simulink model "HapticPaddle_vR2018b"  (R2025a)
settings: Solver=FixedStepAuto  StartTime=0.0  StopTime=10  FixedStep=0.0001  RelTol=1e-3  EnableMultiTasking=on
values from neighbouring files (symbols this model uses):
  B_eq = B_p + R^2*B_m    (= 0.00017775)    [main.m]
  g = 9.81    [main.m]
  J_eq = (J_p + R^2*(J_rotor + J_m))    (= 0.000485304)    [main.m]
  l = 0.0251    [main.m]
  m_p = 0.048    [main.m]
  phi_target = 10.00    (= 10)    [main.m]
  R = r_p1 / r_m    (= 15)    [main.m]
  r_p2 = 0.081    [main.m]
  Tau_f_dry = 0.00156    [main.m]
libraries: simulink_extras x3, slpidlib x1
settings Model: Creator=jemetzge  LastModifiedBy=tk
settings SolverCC: AlgebraicLoopSolver=TrustRegion
settings DataIOCC: LimitDataPoints=on  SaveFormat=Array  SignalLoggingSaveFormat=ModelDataLogs  ReturnWorkspaceOutputs=off
settings OptimizationCC: ExpressionDepthLimit=2147483647.0  LifeSpan=inf
settings DebuggingCC: UnderspecifiedInitializationDetection=Classic  MergeDetectMultiDrivingBlocksExec=none  SolverPrmCheckMsg=warning  FcnCallInpInsideContextMsg=warning  UnconnectedInputMsg=warning  UnconnectedOutputMsg=warning  UnconnectedLineMsg=warning  StateNameClashWarn=warning  SFUnexpectedBacktrackingDiag=warning  SFNoUnconditionalDefaultTransitionDiag=warning  SFExecutionAtInitializationDiag=none  ArithmeticOperatorsInVariantConditions=warning
settings HardwareCC: ProdBitPerPointer=32.0  ProdBitPerSizeT=32.0  ProdBitPerPtrDiffT=32.0  ProdLargestAtomicFloat=None  ProdIntDivRoundTo=Undefined  ProdEndianess=Unspecified  ProdWordSize=32.0  ProdHWDeviceType=32-bit Generic
settings ModelReferenceCC: EnableRefExpFcnMdlSchedulingChecks=on  PropagateSignalLabelsOutOfModel=off
settings SFSimCC: SimUseLocalCustomCode=off  CustomCodeUndefinedFunction=UseInterfaceOnly
settings RTWCC: RTWUseLocalCustomCode=off  GPUComputeCapability=3.5  DLArmComputeVersion=19.05
settings CodeAppCC: StateflowObjectComments=on
settings GRTTargetCC: TargetLangStandard=C89/C90 (ANSI)  CombineOutputUpdateFcns=off  GRTInterface=on
settings ConfigComp: CovMetricSettings=dw  CovSaveCumulativeToWorkspaceVar=on  CovSaveSingleToWorkspaceVar=on  CovExternalEMLEnable=off  CovSFcnEnable=off

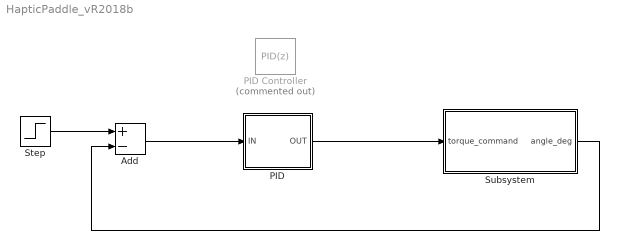
== system HapticPaddle_vR2018b ==
  Add : Sum  Inputs=+-
  PID : Subsystem
  PID Controller : slpidlib/PID Controller  Commented=on  Controller=PID  Form=Parallel  TimeDomain=Discrete-time  UseExternalTs=off  SampleTime=-1  IntegratorMethod=Forward Euler  FilterMethod=Forward Euler  ControllerParametersSource=internal  P=5  I=1  UseKiTs=off  D=5  UseExternalDerivativeSource=off  N=100  UseFilter=on  TunerSelectOption=Transfer Function Based (PID Tuner App)  InitialConditionSource=internal  InitialConditionForIntegrator=0  InitialConditionForFilter=0  DifferentiatorICPrevScaledInput=0  ExternalReset=none  TrackingMode=off  Kt=1  LimitOutput=off  SatLimitsSource=internal  UpperSaturationLimit=inf  LowerSaturationLimit=-inf  LinearizeAsGain=on  AntiWindupMode=none  Kb=1  LimitIntegrator=off  UpperIntegratorSaturationLimit=inf  LowerIntegratorSaturationLimit=-inf  POutMin=[]  POutMax=[]  IOutMin=[]  IOutMax=[]  DOutMin=[]  DOutMax=[]  NOutMin=[]  NOutMax=[]  SumOutMin=[]  SumOutMax=[]  SaturationOutMin=[]  SaturationOutMax=[]  PParamMin=[]  PParamMax=[]  IParamMin=[]  IParamMax=[]  DParamMin=[]  DParamMax=[]  NParamMin=[]  NParamMax=[]  KbParamMin=[]  KbParamMax=[]  KtParamMin=[]  KtParamMax=[]  KbOutMin=[]  KbOutMax=[]  KtOutMin=[]  KtOutMax=[]  IntegratorOutMin=[]  IntegratorOutMax=[]  FilterOutMin=[]  FilterOutMax=[]  SumI1OutMin=[]  SumI1OutMax=[]  SumI2OutMin=[]  SumI2OutMax=[]  SumI3OutMin=[]  SumI3OutMax=[]  SumI4OutMin=[]  SumI4OutMax=[]  SumDOutMin=[]  SumDOutMax=[]  DifferentiatorOutMin=[]  DifferentiatorOutMax=[]  FilterDiffOutCoefMin=[]  FilterDiffOutCoefMax=[]  ReciprocalOutMin=[]  ReciprocalOutMax=[]  SumDenOutMin=[]  SumDenOutMax=[]  SumNumOutMin=[]  SumNumOutMax=[]  DivideOutMin=[]  DivideOutMax=[]  UdiffTsProdOutMin=[]  UdiffTsProdOutMax=[]  NTsProdOutMin=[]  NTsProdOutMax=[]  UintegralTsProdOutMin=[]  UintegralTsProdOutMax=[]  UngainTsProdOutMin=[]  UngainTsProdOutMax=[]  ClampingZeroOutDataTypeStr=Inherit: Inherit via back propagation  ClampingZeroOutMin=[]  ClampingZeroOutMax=[]  FilterDenConstantOutDataTypeStr=Inherit: Inherit via back propagation  FilterDenConstantOutMin=[]  FilterDenConstantOutMax=[]  PCopyOutDataTypeStr=Inherit: Inherit via back propagation  PCopyOutMin=[]  PCopyOutMax=[]  NCopyOutDataTypeStr=Inherit: Inherit via back propagation  NCopyOutMin=[]  NCopyOutMax=[]  IntegratorContinuousStateAttributes=''  IntegratorStateMustResolveToSignalObject=off  IntegratorRTWStateStorageClass=Auto  FilterContinuousStateAttributes=''  FilterStateMustResolveToSignalObject=off  FilterRTWStateStorageClass=Auto  ParallelPVariant=InternalParameters  IdealPVariant=Disabled  IVariant=InternalParameters  DVariant=InternalParameters  IntegratorVariant=Discrete  SatVariant=Disabled  AWVariant=Passthrough  PCopyVariant=Disabled  TRVariant=Disabled  FdbkBlocksVariant=Forward  IdealPFdbkVariant=Disabled  SatFdbkVariant=Disabled  DerivativeFilterVariant=ForwardEulerFilter  NVariant=InternalParameters  NCopyVariant=Disabled  FilterICVariant=InternalICsFilter  IntegratorICVariant=InternalICs  ExternalResetVariant=Disabled  TRSumVariant=Passthrough  SumFdbkVariant=Disabled  SumVariant=Sum_PID  TsampFilterVariant=InternalTs  TsampNgainVariant=Passthrough  TsampIntegralVariant=Disabled_SignalSpec  ExternalSaturationOutDataTypeStr=Inherit: Same as second input  DerivativeSourceVariant=ErrorSignal  PreIntVariant=InternalPreInt
  Step : Step  After=phi_target  SampleTime=0
  Subsystem : Subsystem
  wires:
  PID/1(OUT) -> Subsystem/1(torque_command)
  Subsystem/1(angle_deg) -> Add/2
  Step/1 -> Add/1
  Add/1 -> PID/1(IN)

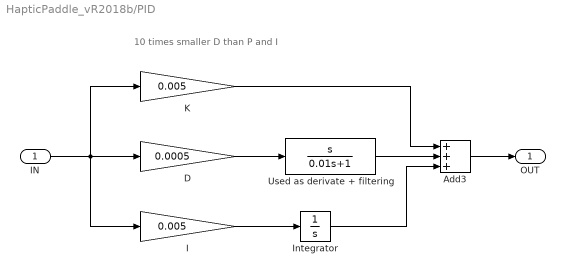
== system HapticPaddle_vR2018b/PID ==
  note: 10 times smaller D than P and I
  IN : Inport
  Add3 : Sum  Inputs=+++
  D : Gain  Gain=0.0005
  I : Gain  Gain=0.005
  Integrator : Integrator
  K : Gain  Gain=0.005
  Used as derivate + filtering : TransferFcn  Numerator=[1 0]  Denominator=[0.01 1]
  OUT : Outport
  wires:
  Integrator/1 -> Add3/3
  I/1 -> Integrator/1
  K/1 -> Add3/1
  Add3/1 -> OUT/1
  D/1 -> Used as derivate + filtering/1
  Used as derivate + filtering/1 -> Add3/2
  IN/1 -> I/1, D/1, K/1

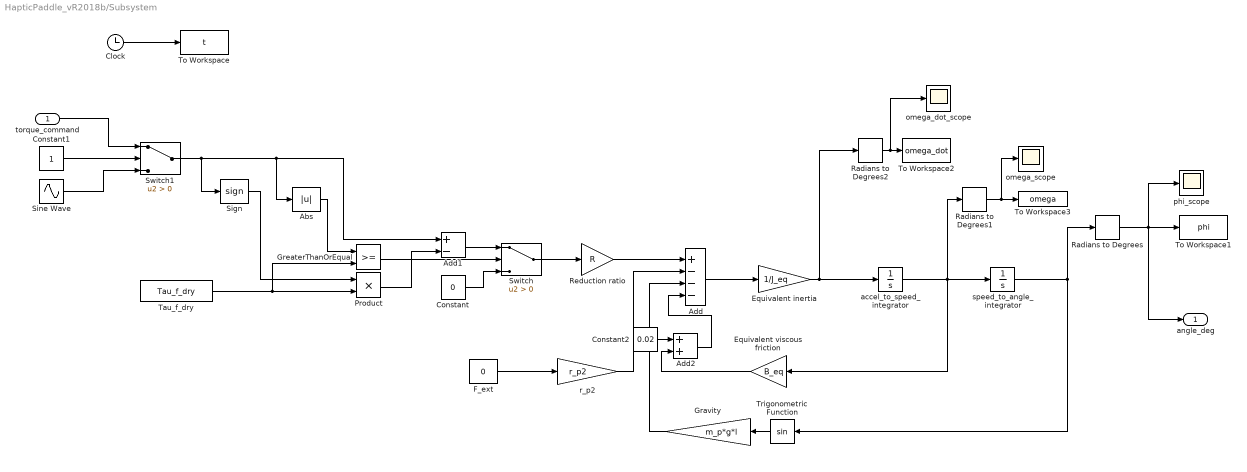
== system HapticPaddle_vR2018b/Subsystem ==
  torque_command : Inport
  Abs : Abs  SaturateOnIntegerOverflow=off
  Add : Sum  Inputs=+---
  Add1 : Sum  Inputs=+-
  Add2 : Sum
  Clock : Clock
  Constant : Constant  Value=0
  Constant1 : Constant
  Constant2 : Constant  Value=0.02
  Equivalent inertia : Gain  Gain=1/J_eq
  Equivalent viscous friction : Gain  Gain=B_eq
  F_ext : Constant  Value=0
  Gravity : Gain  Gain=m_p*g*l
  GreaterThanOrEqual : RelationalOperator  OutDataTypeStr=boolean  RndMeth=Simplest  InputSameDT=off
  Product : Product
  Radians to Degrees : simulink_extras/Transformations/Radians to Degrees
  Radians to Degrees1 : simulink_extras/Transformations/Radians to Degrees
  Radians to Degrees2 : simulink_extras/Transformations/Radians to Degrees
  Reduction ratio : Gain  Gain=R
  Sign : Signum
  Sine Wave : Sin  Amplitude=0.005  Frequency=2*pi*0.5  SampleTime=0
  Switch : Switch  Criteria=u2 > Threshold  SaturateOnIntegerOverflow=off  InputSameDT=off
  Switch1 : Switch  Criteria=u2 > Threshold  SaturateOnIntegerOverflow=off  InputSameDT=off
  Tau_f_dry : Constant  Value=Tau_f_dry
  To Workspace : ToWorkspace  VariableName=t  SampleTime=-1
  To Workspace1 : ToWorkspace  VariableName=phi  SampleTime=-1
  To Workspace2 : ToWorkspace  VariableName=omega_dot  SampleTime=-1
  To Workspace3 : ToWorkspace  VariableName=omega  SampleTime=-1
  Trigonometric Function : Trigonometry
  accel_to_speed_integrator : Integrator
  omega_dot_scope : Scope
      settings: ActiveDisplayYMinimum=-665.97662  ActiveDisplayYMaximum=1557.76798  DataLoggingVariableName=ScopeData2
  omega_scope : Scope
      settings: ActiveDisplayYMinimum=-32.47763  ActiveDisplayYMaximum=185.55824
  phi_scope : Scope
      settings: TimeSpan=10  ActiveDisplayYMinimum=-31.841471785634429  ActiveDisplayYMaximum=0.78130096994778642
  r_p2 : Gain  Gain=r_p2
  speed_to_angle_integrator : Integrator
  angle_deg : Outport
  wires:
  Switch/1 -> Reduction ratio/1
  Clock/1 -> To Workspace/1
  Abs/1 -> GreaterThanOrEqual/1
  Radians to Degrees/1 -> angle_deg/1, phi_scope/1, To Workspace1/1
  Sine Wave/1 -> Switch1/3
  Tau_f_dry/1 -> Product/2, GreaterThanOrEqual/2
  Gravity/1 -> Add/3
  Radians to Degrees2/1 -> omega_dot_scope/1, To Workspace2/1
  Constant1/1 -> Switch1/2
  GreaterThanOrEqual/1 -> Switch/2
  Reduction ratio/1 -> Add/1
  Constant/1 -> Switch/3
  Equivalent inertia/1 -> accel_to_speed_integrator/1, Radians to Degrees2/1
  r_p2/1 -> Add/2
  Radians to Degrees1/1 -> omega_scope/1, To Workspace3/1
  Trigonometric Function/1 -> Gravity/1
  Product/1 -> Add1/2
  Switch1/1 -> Add1/1, Abs/1, Sign/1
  Add/1 -> Equivalent inertia/1
  torque_command/1 -> Switch1/1
  Sign/1 -> Product/1
  speed_to_angle_integrator/1 -> Trigonometric Function/1, Radians to Degrees/1
  Add1/1 -> Switch/1
  accel_to_speed_integrator/1 -> Equivalent viscous friction/1, Radians to Degrees1/1, speed_to_angle_integrator/1
  Equivalent viscous friction/1 -> Add2/2
  F_ext/1 -> r_p2/1
  Add2/1 -> Add/4
  Constant2/1 -> Add2/1
